simulink library "AFCToolbox2023a"  (R2023a)
settings: Solver=VariableStepAuto  StartTime=0.0  StopTime=10.0  RelTol=1e-3
undefined symbols (not defined in the file or in its folder): AFC5Toolbox_SimuMoudle, AFCToolbox, ax, ay, az, btnSample, C_d, C_dm, C_m, C_t, Control, d, declination_table, dp0, dp1, dp2, dp3, dt, euler_0, g0, I_xyz, inclination_table, J_m, lmd_high, lmd_low, lp_acc_knoise, lp_acc_max, lp_acc_min, lp_acc_seed, lp_GPS_BL_max, lp_GPS_BL_min, lp_GPS_H_max, lp_GPS_H_min, lp_GPS_knoise, lp_GPS_seed, lp_GPS_vel_max, lp_GPS_vel_min, lp_gyro_knoise, lp_gyro_max, lp_gyro_min, lp_gyro_seed, lp_hf_vwind, lp_hs_vwind_interp, lp_kaerorho, lp_kaeroT, lp_kIxyz, lp_kmass, lp_momentx_A0, lp_momentx_Af, lp_momentx_ts, lp_momenty_A0, lp_momenty_Af, lp_momenty_ts, lp_momentz_A0, lp_momentz_Af, lp_momentz_ts, lp_vf_vwind, lp_vs_vwind_interp, lp_vwind_thetax, lp_vwind_thetaz ... (+54)
libraries: $bdroot x104, simulink x75, etargetslib x32, sharedtransform x13, simulink_extras x12, dspstat3 x11, aerolibconvert2 x9, aerolibtransform2 x3, aerolibutil x2, matrix_library x1
(part 8 of 10)

== matlab function AFCToolbox2023a/ServoCardModule/XSrvoSamp/MATLAB Function ==
  data: ID1 input; out1 output; angleACK1 input; ID2 input; angleACK2 input; ID3 input; angleACK3 input; ID4 input; angleACK4 input; out2 output; out3 output; out4 output
function [out1, out2, out3, out4] = routeByID(ID1, angleACK1, ID2, angleACK2, ID3, angleACK3, ID4, angleACK4)
    % 1. 初始化输出数组（4个元素，对应Mux1-4号端口，默认0）
    out_array = zeros(1, 4);  % [out1, out2, out3, out4]
    
    % 2. 打包所有ID和angleACK为数组（批量处理，避免重复代码）
    IDs = [ID1, ID2, ID3, ID4];          % 所有ID的数组
    angles = [angleACK1, angleACK2, angleACK3, angleACK4];  % 所有角度的数组
    
    % 3. 循环遍历：ID在1-4范围内才赋值（索引直接对应端口）
    for i = 1:4
        id = IDs(i);
        if id >= 1 && id <= 4  % 仅处理合法ID（1-4）
            out_array(id) = angles(i);  % 关键：ID=1→out_array(1)=out1，直接索引赋值！
        end
    end
    
    % 4. 拆分输出数组为4个端口（对应Mux1-4号）
    [out1, out2, out3, out4] = deal(out_array(1), out_array(2), out_array(3), out_array(4));
end

== matlab function AFCToolbox2023a/SimuMoudle/Position-Control/Consistent formation control /一致性控制——F2/MATLAB Function1 ==
  data: r input; result output
function result = Faixy(r)
%UNTITLED 此处显示有关此函数的摘要


result=-1.8*(1-exp(-0.5*r))/(1+exp(-0.5*r));



end

== matlab function AFCToolbox2023a/SimuMoudle/Position-Control/Consistent formation control /一致性控制——F3/MATLAB Function2 ==
  data: r input; result output
function result = Faixy(r)
%UNTITLED 此处显示有关此函数的摘要


result=-1.8*(1-exp(-0.5*r))/(1+exp(-0.5*r));



end

== matlab function AFCToolbox2023a/SimuMoudle/Position-Control/Consistent formation control /一致性控制——F1/Subsystem1/MATLAB Function ==
  data: i input; wx output; dt input; wy output
function [wx,wy] = w_error(i,dt)
%W_ERROR 此处显示有关此函数的摘要
%   此处显示详细说明
wx = 0.1*(cos(i*dt+pi/6)+cos(i*dt/3+pi/6)+cos(i*dt/5+pi/6)+cos(i*dt/7+pi/6));
wy = 0.1*(sin(i*dt+pi/6)+sin(i*dt/3+pi/6)+sin(i*dt/5+pi/6)+sin(i*dt/7+pi/6));

end

== matlab function AFCToolbox2023a/SimuMoudle/Position-Control/Consistent formation control /一致性控制——F2/Subsystem2/MATLAB Function ==
  data: i input; wx output; dt input; wy output
function [wx,wy] = w_error(i,dt)
%W_ERROR 此处显示有关此函数的摘要
%   此处显示详细说明
wx = 0.1*(cos(i*dt+pi/6)+cos(i*dt/3+pi/6)+cos(i*dt/5+pi/6)+cos(i*dt/7+pi/6));
wy = 0.1*(sin(i*dt+pi/6)+sin(i*dt/3+pi/6)+sin(i*dt/5+pi/6)+sin(i*dt/7+pi/6));

end

== matlab function AFCToolbox2023a/SimuMoudle/Position-Control/Consistent formation control /一致性控制——F3/Subsystem1/MATLAB Function ==
  data: i input; wx output; dt input; wy output
function [wx,wy] = w_error(i,dt)
%W_ERROR 此处显示有关此函数的摘要
%   此处显示详细说明
wx = 0.1*(cos(i*dt+pi/6)+cos(i*dt/3+pi/6)+cos(i*dt/5+pi/6)+cos(i*dt/7+pi/6));
wy = 0.1*(sin(i*dt+pi/6)+sin(i*dt/3+pi/6)+sin(i*dt/5+pi/6)+sin(i*dt/7+pi/6));

end

== matlab function AFCToolbox2023a/SimuMoudle/Position-Control/Consistent formation control /一致性控制——F2/MATLAB Function2 ==
  data: r input; result output
function result = Faixy(r)
%UNTITLED 此处显示有关此函数的摘要


result=-1.8*(1-exp(-0.5*r))/(1+exp(-0.5*r));



end

== matlab function AFCToolbox2023a/SimuMoudle/Position-Control/Consistent formation control /一致性控制——F1/MATLAB Function1 ==
  data: r input; result output
function result = Faixy(r)
%UNTITLED 此处显示有关此函数的摘要


result=-1.8*(1-exp(-0.5*r))/(1+exp(-0.5*r));



end

== matlab function AFCToolbox2023a/SimuMoudle/Position-Control/Consistent formation control /一致性控制——F1/MATLAB Function2 ==
  data: r input; result output
function result = Faixy(r)
%UNTITLED 此处显示有关此函数的摘要


result=-1.8*(1-exp(-0.5*r))/(1+exp(-0.5*r));



end

== matlab function AFCToolbox2023a/SimuMoudle/Position-Control/Consistent formation control /一致性控制——F1/MATLAB Function4 ==
  data: r input; result output
function result = Faixy(r)
%UNTITLED 此处显示有关此函数的摘要


result=-1.8*(1-exp(-0.5*r))/(1+exp(-0.5*r));



end

== matlab function AFCToolbox2023a/SimuMoudle/Position-Control/Consistent formation control /一致性控制——F3/MATLAB Function3 ==
  data: r input; result output
function result = Faixy(r)
%UNTITLED 此处显示有关此函数的摘要


result=-1.8*(1-exp(-0.5*r))/(1+exp(-0.5*r));



end

== matlab function AFCToolbox2023a/SimuMoudle/Position-Control/Leader/Subsystem/Follower1/MATLAB Function ==
  data: theta input; J output; phi input; v input
function J = TA_xyz(theta,phi,v)
a=cos(theta)*cos(phi);
b=-v*sin(theta)*cos(phi);
c=-v*cos(theta)*sin(phi);

d=sin(theta)*cos(phi);
e=v*cos(theta)*cos(phi);
f=-v*sin(theta)*sin(phi);

g=sin(phi);
h=0;
i=v*cos(phi);

J=[a,b,c;
    d,e,f;
    g,h,i];
end

== matlab function AFCToolbox2023a/SimuMoudle/Position-Control/Leader/Subsystem/Follower1/MATLAB Function1 ==
  data: W input; result output
function result = Faiv(W)
%UNTITLED 此处显示有关此函数的摘要


result=-0.5*(1-exp(-0.5*W))/(1+exp(-0.5*W));



end

== matlab function AFCToolbox2023a/SimuMoudle/Position-Control/Leader/Subsystem/Follower1/MATLAB Function2 ==
  data: w input; result output
function result = Faiv(w)
%UNTITLED 此处显示有关此函数的摘要


result=-0.5*(1-exp(-0.5*w))/(1+exp(-0.5*w));



end

== matlab function AFCToolbox2023a/SimuMoudle/Position-Control/Leader/Subsystem/Follower1/MATLAB Function3 ==
  data: r input; result output
function result = Faiv(r)
%UNTITLED 此处显示有关此函数的摘要


result=-0.5*(1-exp(-0.5*r))/(1+exp(-0.5*r));



end

== matlab function AFCToolbox2023a/SimuMoudle/Position-Control/Leader/Subsystem/Follower2/MATLAB Function ==
  data: theta input; J output; phi input; v input
function J = TA_xyz(theta,phi,v)
a=cos(theta)*cos(phi);
b=-v*sin(theta)*cos(phi);
c=-v*cos(theta)*sin(phi);

d=sin(theta)*cos(phi);
e=v*cos(theta)*cos(phi);
f=-v*sin(theta)*sin(phi);

g=sin(phi);
h=0;
i=v*cos(phi);

J=[a,b,c;
    d,e,f;
    g,h,i];
end

== matlab function AFCToolbox2023a/SimuMoudle/Position-Control/Leader/Subsystem/Follower2/MATLAB Function1 ==
  data: W input; result output
function result = Faiv(W)
%UNTITLED 此处显示有关此函数的摘要


result=-0.5*(1-exp(-0.5*W))/(1+exp(-0.5*W));



end

== matlab function AFCToolbox2023a/SimuMoudle/Position-Control/Leader/Subsystem/Follower2/MATLAB Function2 ==
  data: w input; result output
function result = Faiv(w)
%UNTITLED 此处显示有关此函数的摘要


result=-0.5*(1-exp(-0.5*w))/(1+exp(-0.5*w));



end

== matlab function AFCToolbox2023a/SimuMoudle/Position-Control/Leader/Subsystem/Follower2/MATLAB Function3 ==
  data: r input; result output
function result = Faiv(r)
%UNTITLED 此处显示有关此函数的摘要


result=-0.5*(1-exp(-0.5*r))/(1+exp(-0.5*r));



end

== matlab function AFCToolbox2023a/SimuMoudle/Position-Control/Leader/Subsystem/Follower3/MATLAB Function ==
  data: theta input; J output; phi input; v input
function J = TA_xyz(theta,phi,v)
a=cos(theta)*cos(phi);
b=-v*sin(theta)*cos(phi);
c=-v*cos(theta)*sin(phi);

d=sin(theta)*cos(phi);
e=v*cos(theta)*cos(phi);
f=-v*sin(theta)*sin(phi);

g=sin(phi);
h=0;
i=v*cos(phi);

J=[a,b,c;
    d,e,f;
    g,h,i];
end

== matlab function AFCToolbox2023a/SimuMoudle/Position-Control/Leader/Subsystem/Follower3/MATLAB Function1 ==
  data: W input; result output
function result = Faiv(W)
%UNTITLED 此处显示有关此函数的摘要


result=-0.5*(1-exp(-0.5*W))/(1+exp(-0.5*W));



end

== stateflow chart AFCToolbox2023a/SimuMoudle/UAV/Equations of Motion/Chart ==
  state Land
    en, du: ground_contact = 1;
  state Flight
    en, du: ground_contact = 0;
  (default) -> Land
  Flight -> Land : [h<=0 && vel(3) >0]
  Land -> Flight : [acc(3)<0]
  data: h input; vel input; acc input; ground_contact output

== matlab function AFCToolbox2023a/SimuMoudle/Position-Control/Leader/Subsystem/Follower3/MATLAB Function2 ==
  data: w input; result output
function result = Faiv(w)
%UNTITLED 此处显示有关此函数的摘要


result=-0.5*(1-exp(-0.5*w))/(1+exp(-0.5*w));



end

== matlab function AFCToolbox2023a/SimuMoudle/Position-Control/Leader/Subsystem/Follower3/MATLAB Function3 ==
  data: r input; result output
function result = Faiv(r)
%UNTITLED 此处显示有关此函数的摘要


result=-0.5*(1-exp(-0.5*r))/(1+exp(-0.5*r));



end

== matlab function AFCToolbox2023a/SimuMoudle/SimuGps/LLA model/Subsystem1/ECEF地心坐标系-经纬高 ==
  data: x input; l output; y input; z input; b output; h output
function [l,b,h] = fcn(x,y,z)
[l,b,h] = xyz2lbh(x,y,z);

== matlab function AFCToolbox2023a/SimuMoudle/Position-Control/Consistent formation control /一致性控制——F3/MATLAB Function1 ==
  data: r input; result output
function result = Faixy(r)
%UNTITLED 此处显示有关此函数的摘要


result=-1.8*(1-exp(-0.5*r))/(1+exp(-0.5*r));



end

== matlab function AFCToolbox2023a/SimuMoudle/SimuGps/LLA model/Subsystem1/北天东-ECEF地心坐标系 ==
  data: pn input; DX output; ph input; pe input; Lon0 input; Lat0 input; Alt0 input; DY output; DZ output
function [ DX,DY,DZ ] = TransformBTD_T_DX( pn,ph,pe,Lon0,Lat0,Alt0 )
%TransformBTDTDX 此处显示有关此函数的摘要
%将北天东系转换到地心坐标系
m_dN_LE = zeros(3,3);

[ DX0,DY0,DZ0 ] = TransformLLA_T_DX(Lon0,Lat0,Alt0);%经纬高转为地面坐标系G

Fai = Lat0;
Lamda = Lon0;

x_bt = pn;
y_bt = ph;
z_bt = pe;

m_dN_LE(1,1) = -sin(Fai)*cos(Lamda);
m_dN_LE(1,2) = cos(Fai)*cos(Lamda);
m_dN_LE(1,3) = -sin(Lamda);
m_dN_LE(2,1) = -sin(Fai)*sin(Lamda);
m_dN_LE(2,2) = cos(Fai)*sin(Lamda);
m_dN_LE(2,3) = cos(Lamda);
m_dN_LE(3,1) = cos(Fai);
m_dN_LE(3,2) = sin(Fai);
m_dN_LE(3,3) = 0.0;

A = m_dN_LE*[x_bt;y_bt;z_bt];
x_dx = A(1);
y_dx = A(2);
z_dx = A(3);

DX = DX0 + x_dx;
DY = DY0 + y_dx;
DZ = DZ0 + z_dx;

end

== matlab function AFCToolbox2023a/SimuMoudle/SimuICM/acclerate  model2/Subsystem/MATLAB Function ==
  data: accBias input; accData output; correlationTimeConstant input; accNoiseStdDev input; dt input
function accData= fcn(accBias,correlationTimeConstant,accNoiseStdDev,dt)
persistent initaccBias;

%单位换算
arcdeg = pi/180;hur = 3600;dph = arcdeg / hur;Hz = 1;g=9.7803267714;
% accNoiseStdDev = 100;           % 加速度一阶马尔可夫噪声均方根ug
% accBiasOffsetStdDev =100;      % 陀螺仪零偏漂移标准差ug
% 
% %常值漂移
% eb = accBiasOffsetStdDev * g * randn(1,1);

%一阶马尔可夫相关时间T;反相关时间beta = 1/T;
% TauG = 3600;
beta = 1/correlationTimeConstant; 
% 方差R0（m/s^2）
R0 = (accNoiseStdDev*g)^2;

%角速率随机游走系数
q = 2*beta*R0;


if isempty(initaccBias)
    initaccBias = sqrt(R0)*randn(1,1);
    accBias= initaccBias;
end

 
Phi = 1 -beta*dt;
sQkr =sqrt(q*dt);
accBias=Phi*accBias+sQkr*randn(1,1);
% 生成加速度数据
accData =  accBias;
end

== matlab function AFCToolbox2023a/SimuMoudle/SimuICM/acclerate  model2/Subsystem1/MATLAB Function ==
  data: accBias input; accData output; correlationTimeConstant input; accNoiseStdDev input; dt input
function accData= fcn(accBias,correlationTimeConstant,accNoiseStdDev,dt)
persistent initaccBias;

%单位换算
arcdeg = pi/180;hur = 3600;dph = arcdeg / hur;Hz = 1;g=9.7803267714;
% accNoiseStdDev = 100;           % 加速度一阶马尔可夫噪声均方根ug
% accBiasOffsetStdDev =100;      % 陀螺仪零偏漂移标准差ug
% 
% %常值漂移
% eb = accBiasOffsetStdDev * g * randn(1,1);

%一阶马尔可夫相关时间T;反相关时间beta = 1/T;
% TauG = 3600;
beta = 1/correlationTimeConstant; 
% 方差R0（m/s^2）
R0 = (accNoiseStdDev*g)^2;

%角速率随机游走系数
q = 2*beta*R0;


if isempty(initaccBias)
    initaccBias = sqrt(R0)*randn(1,1);
    accBias= initaccBias;
end

 
Phi = 1 -beta*dt;
sQkr =sqrt(q*dt);
accBias=Phi*accBias+sQkr*randn(1,1);
% 生成加速度数据
accData =  accBias;
end

== matlab function AFCToolbox2023a/SimuMoudle/SimuICM/acclerate  model2/Subsystem2/MATLAB Function ==
  data: accBias input; accData output; correlationTimeConstant input; accNoiseStdDev input; dt input
function accData= fcn(accBias,correlationTimeConstant,accNoiseStdDev,dt)
persistent initaccBias;

%单位换算
arcdeg = pi/180;hur = 3600;dph = arcdeg / hur;Hz = 1;g=9.7803267714;
% accNoiseStdDev = 100;           % 加速度一阶马尔可夫噪声均方根ug
% accBiasOffsetStdDev =100;      % 陀螺仪零偏漂移标准差ug
% 
% %常值漂移
% eb = accBiasOffsetStdDev * g * randn(1,1);

%一阶马尔可夫相关时间T;反相关时间beta = 1/T;
% TauG = 3600;
beta = 1/correlationTimeConstant; 
% 方差R0（m/s^2）
R0 = (accNoiseStdDev*g)^2;

%角速率随机游走系数
q = 2*beta*R0;


if isempty(initaccBias)
    initaccBias = sqrt(R0)*randn(1,1);
    accBias= initaccBias;
end

 
Phi = 1 -beta*dt;
sQkr =sqrt(q*dt);
accBias=Phi*accBias+sQkr*randn(1,1);
% 生成加速度数据
accData =  accBias;
end

== matlab function AFCToolbox2023a/SimuMoudle/SimuICM/gyro model1/Subsystem/MATLAB Function ==
  data: gyroBias input; gyroData output; correlationTimeConstant input; gyroNoiseStdDev input; dt input
function gyroData= fcn(gyroBias,correlationTimeConstant,gyroNoiseStdDev,dt)
persistent initgyroBias;

%单位换算
arcdeg = pi/180;hur = 3600;dph = arcdeg / hur;Hz = 1;
% gyroNoiseStdDev = 0.1;           % 陀螺仪一阶马尔可夫噪声均方根°/h
% gyroBiasOffsetStdDev = 0.1;      % 陀螺仪零偏漂移标准差rad/s
% 
% %常值漂移
% eb = gyroBiasOffsetStdDev * dph * randn(1,1);

%一阶马尔可夫相关时间T;反相关时间beta = 1/T;
% TauG = 3600;
beta = 1/correlationTimeConstant; 
% 方差R0（rad/s）
R0 = (gyroNoiseStdDev*dph)^2;

%角速率随机游走系数
q = 2*beta*R0;


if isempty(initgyroBias)
    initgyroBias = sqrt(R0)*randn(1,1);
    gyroBias= initgyroBias;
end

 
Phi = 1 -beta*dt;
sQkr =sqrt(q*dt);
gyroBias=Phi*gyroBias+sQkr*randn(1,1);
% 生成陀螺仪数据
gyroData =  gyroBias;
end

== matlab function AFCToolbox2023a/SimuMoudle/SimuICM/gyro model1/Subsystem1/MATLAB Function ==
  data: gyroBias input; gyroData output; correlationTimeConstant input; gyroNoiseStdDev input; dt input
function gyroData= fcn(gyroBias,correlationTimeConstant,gyroNoiseStdDev,dt)
persistent initgyroBias;

%单位换算
arcdeg = pi/180;hur = 3600;dph = arcdeg / hur;Hz = 1;
% gyroNoiseStdDev = 0.1;           % 陀螺仪一阶马尔可夫噪声均方根°/h
% gyroBiasOffsetStdDev = 0.1;      % 陀螺仪零偏漂移标准差rad/s
% 
% %常值漂移
% eb = gyroBiasOffsetStdDev * dph * randn(1,1);

%一阶马尔可夫相关时间T;反相关时间beta = 1/T;
% TauG = 3600;
beta = 1/correlationTimeConstant; 
% 方差R0（rad/s）
R0 = (gyroNoiseStdDev*dph)^2;

%角速率随机游走系数
q = 2*beta*R0;


if isempty(initgyroBias)
    initgyroBias = sqrt(R0)*randn(1,1);
    gyroBias= initgyroBias;
end

 
Phi = 1 -beta*dt;
sQkr =sqrt(q*dt);
gyroBias=Phi*gyroBias+sQkr*randn(1,1);
% 生成陀螺仪数据
gyroData =  gyroBias;
end

== matlab function AFCToolbox2023a/SimuMoudle/Position-Control/Leader/MATLAB Function ==
  data: theta input; J output; phi input; v input
function J = TA_xyz(theta,phi,v)
a=cos(theta)*cos(phi);
b=-v*sin(theta)*cos(phi);
c=-v*cos(theta)*sin(phi);

d=sin(theta)*cos(phi);
e=v*cos(theta)*cos(phi);
f=-v*sin(theta)*sin(phi);

g=sin(phi);
h=0;
i=v*cos(phi);

J=[a,b,c;
    d,e,f;
    g,h,i];
end

== matlab function AFCToolbox2023a/SimuMoudle/SimuICM/gyro model1/Subsystem2/MATLAB Function ==
  data: gyroBias input; gyroData output; correlationTimeConstant input; gyroNoiseStdDev input; dt input
function gyroData= fcn(gyroBias,correlationTimeConstant,gyroNoiseStdDev,dt)
persistent initgyroBias;

%单位换算
arcdeg = pi/180;hur = 3600;dph = arcdeg / hur;Hz = 1;
% gyroNoiseStdDev = 0.1;           % 陀螺仪一阶马尔可夫噪声均方根°/h
% gyroBiasOffsetStdDev = 0.1;      % 陀螺仪零偏漂移标准差rad/s
% 
% %常值漂移
% eb = gyroBiasOffsetStdDev * dph * randn(1,1);

%一阶马尔可夫相关时间T;反相关时间beta = 1/T;
% TauG = 3600;
beta = 1/correlationTimeConstant; 
% 方差R0（rad/s）
R0 = (gyroNoiseStdDev*dph)^2;

%角速率随机游走系数
q = 2*beta*R0;


if isempty(initgyroBias)
    initgyroBias = sqrt(R0)*randn(1,1);
    gyroBias= initgyroBias;
end

 
Phi = 1 -beta*dt;
sQkr =sqrt(q*dt);
gyroBias=Phi*gyroBias+sQkr*randn(1,1);
% 生成陀螺仪数据
gyroData =  gyroBias;
end

== matlab function AFCToolbox2023a/SimuMoudle/SimuBaro/Baro model/MATLAB Function ==
  data: h input; P output
function P = altitude_to_pressure(h)
    % 输入：高度 h（单位：米）
    % 输出：压强 P（单位：Pa）

    % 常量定义
    P0 = 101325;  % 海平面上的大气压强，单位Pa
    L = 0.0065;   % 温度递减率，单位K/m
    T0 = 288.15;  % 海平面上的温度，单位K
    g0 = 9.80665; % 重力加速度，单位m/s²
    M = 0.0289644; % 空气摩尔质量，单位kg/mol
    R = 8.314462618; % 气体常数，单位J/(mol·K)

    % 计算压强
    P = P0 * (1 - (L * h) / T0)^(g0 * M / (R * L));
end

== matlab function AFCToolbox2023a/SimuMoudle/SimuBaro/Baro model/MATLAB Function1 ==
  data: altitude input; pressure output; temperature output
function [pressure, temperature] = calculateAtmosphereProperties(altitude)
    % 标准大气参数
    R = 287; % 干空气的特定气体常数，单位 J/(kg*K)
    g = 9.81; % 重力加速度，单位 m/s^2
    T0 = 293.15; % 海平面标准温度，单位 K
    p0 = 101325; % 海平面标准压强，单位 Pa
    lapserate = -0.0065; % 环境递减率，单位 K/m

    % 计算给定高度的压强和温度
    if altitude <= 11000
        temperature = T0 + lapserate * altitude; % 温度随高度线性递减
    else
        temperature = T0 + lapserate * 11000; % 高于11公里后温度保持不变
    end
    pressure = p0 * (T0/temperature)^(-g/R/lapserate); % 压强随高度和温度变化

    % 输出结果
    pressure = pressure; % 返回压强
    
    % 将温度从开尔文转换为摄氏度
    temperature = temperature - 273.15;% 返回温度
end

== matlab function AFCToolbox2023a/基础导航算法模型库/ECL EKF/Subsystem/InitCovariance1 ==
  data: covariance output; dt input
function covariance = InitCovariance(dt)
%% Initial Uncertainty
param.alignment.posErrNE = 10.0; % Initial 1SD position error when aligning without GPS. (m/sec)
param.alignment.velErrNE = 5.0; % Initial 1SD velocity error when aligning without GPS. (m/sec)
param.alignment.velErrD = 1.0; % Initial 1SD vertical velocity error when aligning without GPS. (m/sec)
param.alignment.delAngBiasErr = 0.05*pi/180; % Initial 1SD rate gyro bias uncertainty. (rad/sec)
param.alignment.delVelBiasErr = 0.07; % Initial 1SD accelerometer bias uncertainty. (m/sec^2)
param.alignment.quatErr = 0.01; % Initial 1SD uncertainty in quaternion.
param.alignment.magErrXYZ = 0.01; % Initial 1SD uncertainty in body frame XYZ magnetic field states. (gauss)
param.alignment.magErrNED = 0.5; % Initial 1SD uncertainty in earth frame NED magnetic field states. (gauss)
param.alignment.hgtErr = 0.5; % Initial 1SD uncertainty in height. (m)
param.alignment.windErrNE = 5.0; % Initial 1SD error in wind states. (m/sec)


% Define quaternion state errors
Sigma_quat = param.alignment.quatErr * [1;1;1;1];
% Define velocity state errors
Sigma_velocity = param.alignment.velErrNE * [1;1;1];

% Define position state errors
Sigma_position = param.alignment.posErrNE * [1;1;1];


% Define delta angle bias state errors
Sigma_dAngBias = param.alignment.delAngBiasErr*dt*[1;1;1];

% Define delta velocity bias state errors
Sigma_dVelBias = param.alignment.delVelBiasErr*dt*[1;1;1];

% Define magnetic field state errors
Sigma_magNED = [param.alignment.magErrNED;param.alignment.magErrNED;param.alignment.magErrNED]; % 1 Sigma uncertainty in initial NED mag field
Sigma_magXYZ = [param.alignment.magErrXYZ;param.alignment.magErrXYZ;param.alignment.magErrXYZ]; % 1 Sigma uncertainty in initial XYZ mag sensor offset

% Define wind velocity state errors
Sigma_wind = param.alignment.windErrNE * [1;1];

% Convert to variances and write to covariance matrix diagonals
covariance = diag([Sigma_quat;Sigma_velocity;Sigma_position;Sigma_dAngBias;Sigma_dVelBias;Sigma_magNED;Sigma_magXYZ;Sigma_wind].^2);
end

== matlab function AFCToolbox2023a/基础导航算法模型库/ECL EKF/Subsystem/Mag Fusion/Control MagDeclination Fusion1 ==
  data: states input; states output; P input; R_decl input; measDec input; P output
function [...
    states, ... % state vector after fusion of measurements
    P] ... %
    = FuseMagDeclination( ...
    states, ... % state vector after fusion of measurements
    P, ... %
    R_decl,...
    measDec) % magnetic field declination - azimuth angle measured from true north (rad)

% magNE
magN = states(17);
magE = states(18);

H = zeros(1,24);
Kfusion = zeros(24,1);

R_DECL = R_decl^2;
	HK0 = power(magN, -2);
	HK1 = HK0*power(magE, 2) + 1.0;
	HK2 = 1.0/HK1;
	HK3 = 1.0/magN;
	HK4 = HK2*HK3;
    HK5 = HK3*magE;
	HK6 = HK5*P(17,18) - P(18,18);
	HK7 = power(HK1, -2);
	HK8 = HK5*P(17,17) - P(17,18);
    innovation_variance = -HK0*HK6*HK7 + HK7*HK8*magE/power(magN, 3) + R_DECL;
    HK9 = HK4/innovation_variance;

H(17) = -HK0*HK2*magE;
H(18) = HK4;

	for row = 1:16
		Kfusion(row) = -HK9*(HK5*P(row,17) - P(row,18));
    end

	Kfusion(17) = -HK8*HK9;
	Kfusion(18) = -HK6*HK9;

	for  row = 19:24
		Kfusion(row) = -HK9*(HK5*P(17,row) - P(18,row));
    end


% Magnetic declination noise R = σdelc^2
%R_MAG = 0.5^2;

%% Hψ_dec = ∂ψ_dec / ∂x
%H = calcH_MAGD(magE,magN);
% S = Hψ_dec * P * PT + R_MAG
%varInnov = (H*P*transpose(H) + R_MAG);
% Optimal Kalman gain, K = Pk+1|k * Hψ_dec / S
%Kfusion = (P*transpose(H))/varInnov;

% Calculate the predicted magnetic declination, ψ_dec = arctan(mE/mN)
predDec = atan2(magE,magN);

% Calculate the measurement innovation, yk = zψ_dec - ψ_dec
innovation = measDec- predDec;

if (innovation > 0.5)
    innovation = single(0.5);
elseif (innovation < -0.5)
    innovation = single(-0.5);
end

% correct the state vector, xk+1|k+1 = xk+1|k + K*yk
states = states + Kfusion * innovation;

% correct the covariance Pk+1|k+1 = Pk+1|k - K * Hψ_dec * Pk+1|k
%P = P - Kfusion*H*P;
KHP = computeKHP(Kfusion, H, P);
P = P - KHP;
%% Force symmetry on the covariance matrix to prevent ill-conditioning
% of the matrix which would cause the filter to blow-up
P = 0.5*(P + transpose(P));

% ensure diagonals are positive
for i=1:24
    if P(i,i) < 0
        P(i,i) = single(0);
    end
end
% fixCovarianceErrors(true);
% limitDeclination();
end

== matlab function AFCToolbox2023a/基础导航算法模型库/ECL EKF/Subsystem/Mag Fusion/Control Magneto meter Fusion2 ==
  data: fault_status_flags_bad_mag output; states input; states output; P input; Measmag input; R_MAG input; P output
function [fault_status_flags_bad_mag,...
    states, ... % state vector after fusion of measurements
    P] ...% state covariance matrix after fusion of corrections
    = FuseMagnetometer( ...
    states, ... % predicted states
    P, ... % predicted covariance
    Measmag, ... % body frame magnetic flux measurements
    R_MAG) % magnetometer measurement variance - gauss^2
   
% control.cpp -> controlMagFusion()
% ~ mag_control.cpp -> controlMagFusion() -> runMagAndMagDeclFusions(...)-> 
% ~ mag_fusion.cpp -> fuseMag(...) -> fuseDeclination(...)
fault_status_flags_bad_mag = zeros(1,3);
% assign intermediate variables

% quaternion
q0 = states(1);
q1 = states(2);
q2 = states(3);
q3 = states(4);
% magnetometer bais
magXbias = states(20);
magYbias = states(21);
magZbias = states(22);
mag_B = [magXbias;magYbias;magZbias];
% magNED
magN = states(17);
magE = states(18);
magD = states(19);


% XYZ Measurement uncertainty. Need to consider timing errors for fast rotations
% R_MAG = power(max(params_mag_noise, 0.0),2);
mag_innov_var = zeros(1,3);

% calculate intermediate variables used for X axis innovation variance, observation Jacobians and Kalman gains
% const char* numerical_error_covariance_reset_string = "numerical error - covariance reset";
HKX0 = -magD*q2 + magE*q3 + magN*q0;
HKX1 = magD*q3 + magE*q2 + magN*q1;
HKX2 = magE*q1;
HKX3 = magD*q0;
HKX4 = magN*q2;
HKX5 = magD*q1 + magE*q0 - magN*q3;
HKX6 = power(q0, 2) + power(q1, 2) - power(q2, 2) - power(q3, 2);
HKX7 = q0*q3 + q1*q2;
HKX8 = q1*q3;
HKX9 = q0*q2;
HKX10 = 2*HKX7;
HKX11 = -2*HKX8 + 2*HKX9;
HKX12 = 2*HKX1;
HKX13 = 2*HKX0;
HKX14 = -2*HKX2 + 2*HKX3 + 2*HKX4;
HKX15 = 2*HKX5;
HKX16 = HKX10*P(1,18) - HKX11*P(1,19) + HKX12*P(1,2) + HKX13*P(1,1) - HKX14*P(1,3) + HKX15*P(1,4) + HKX6*P(1,17) + P(1,20);
HKX17 = HKX10*P(17,18) - HKX11*P(17,19) + HKX12*P(2,17) + HKX13*P(1,17) - HKX14*P(3,17) + HKX15*P(4,17) + HKX6*P(17,17) + P(17,18);
HKX18 = HKX10*P(18,19) - HKX11*P(19,19) + HKX12*P(2,19) + HKX13*P(1,19) - HKX14*P(3,19) + HKX15*P(4,19) + HKX6*P(17,19) + P(19,20);
HKX19 = HKX10*P(3,18) - HKX11*P(3,19) + HKX12*P(2,3) + HKX13*P(1,3) - HKX14*P(3,3) + HKX15*P(3,4) + HKX6*P(3,17) + P(3,20);
HKX20 = HKX10*P(18,18) - HKX11*P(18,19) + HKX12*P(2,18) + HKX13*P(1,18) - HKX14*P(3,18) + HKX15*P(4,18) + HKX6*P(17,18) + P(18,20);
HKX21 = HKX10*P(4,18) - HKX11*P(4,19) + HKX12*P(2,4) + HKX13*P(1,4) - HKX14*P(3,4) + HKX15*P(4,4) + HKX6*P(4,17) + P(4,20);
HKX22 = HKX10*P(2,18) - HKX11*P(2,19) + HKX12*P(2,2) + HKX13*P(1,2) - HKX14*P(2,3) + HKX15*P(2,4) + HKX6*P(2,17) + P(2,20);
HKX23 = HKX10*P(18,20) - HKX11*P(19,20) + HKX12*P(2,20) + HKX13*P(1,20) - HKX14*P(3,20) + HKX15*P(4,20) + HKX6*P(17,20) + P(20,20);

mag_innov_var(1) = HKX10*HKX20 - HKX11*HKX18 + HKX12*HKX22 + HKX13*HKX16 - HKX14*HKX19 + HKX15*HKX21 + HKX17*HKX6 + HKX23 + R_MAG;

if (mag_innov_var(1) < R_MAG) 
	% the innovation variance contribution from the state covariances is negative which means the covariance matrix is badly conditioned
	fault_status_flags_bad_mag_x = 1;

	% we need to re-initialise covariances and abort this fusion step
	% resetMagRelatedCovariances();
    P = resetMagRelatedCovariances(P,states);
    return;
end
fault_status_flags_bad_mag_x = 0;
% fault_status_flags_bad_mag_x = false;

HKX24 = 1.0/mag_innov_var(1);

% intermediate variables for calculation of innovations variances for Y and Z axes
% don't calculate all terms needed for observation jacobians and Kalman gains because
% these will have to be recalculated when the X and Y axes are fused
IV0 = q0*q1;
IV1 = q2*q3;
IV2 = 2*IV0 + 2*IV1;
IV3 = 2*q0*q3 - 2*q1*q2;
IV4 = 2*magD*q3 + 2*magE*q2 + 2*magN*q1;
IV5 = 2*magD*q1 + 2*magE*q0 - 2*magN*q3;
IV6 = 2*magD*q0 - 2*magE*q1 + 2*magN*q2;
IV7 = -2*magD*q2 + 2*magE*q3 + 2*magN*q0;
IV8 = power(q2, 2);
IV9 = power(q3, 2);
IV10 = power(q0, 2) - power(q1, 2);
IV11 = IV10 + IV8 - IV9;
% const float IV12 = IV7*P(2,3);
% const float IV13 = IV5*P(0,1);
% const float IV14 = IV6*P(0,1);
% const float IV15 = IV4*P(2,3);
IV12 = IV7*P(3,4);
IV13 = IV5*P(1,2);
IV14 = IV6*P(1,2);
IV15 = IV4*P(3,4);
IV16 = 2*q0*q2 + 2*q1*q3;
IV17 = 2*IV0 - 2*IV1;
IV18 = IV10 - IV8 + IV9;
% _mag_innov_var(1) = IV11*P(17,20) + IV11*(IV11*P(17,17) + IV2*P(17,18) - IV3*P(16,17) + IV4*P(2,17) + IV5*P(0,17) + IV6*P(1,17) - IV7*P(3,17) + P(17,20)) + IV2*P(18,20) + IV2*(IV11*P(17,18) + IV2*P(18,18) - IV3*P(16,18) + IV4*P(2,18) + IV5*P(0,18) + IV6*P(1,18) - IV7*P(3,18) + P(18,20)) - IV3*P(16,20) - IV3*(IV11*P(16,17) + IV2*P(16,18) - IV3*P(16,16) + IV4*P(2,16) + IV5*P(0,16) + IV6*P(1,16) - IV7*P(3,16) + P(16,20)) + IV4*P(2,20) + IV4*(IV11*P(2,17) - IV12 + IV2*P(2,18) - IV3*P(2,16) + IV4*P(2,2) + IV5*P(0,2) + IV6*P(1,2) + P(2,20)) + IV5*P(0,20) + IV5*(IV11*P(0,17) + IV14 + IV2*P(0,18) - IV3*P(0,16) + IV4*P(0,2) + IV5*P(0,0) - IV7*P(0,3) + P(0,20)) + IV6*P(1,20) + IV6*(IV11*P(1,17) + IV13 + IV2*P(1,18) - IV3*P(1,16) + IV4*P(1,2) + IV6*P(1,1) - IV7*P(1,3) + P(1,20)) - IV7*P(3,20) - IV7*(IV11*P(3,17) + IV15 + IV2*P(3,18) - IV3*P(3,16) + IV5*P(0,3) + IV6*P(1,3) - IV7*P(3,3) + P(3,20)) + P(20,20) + R_MAG;
mag_innov_var(2) = IV11*P(18,21) + IV11*(IV11*P(18,18) + IV2*P(18,19) - IV3*P(17,18) + IV4*P(3,18) + IV5*P(1,18) + IV6*P(2,18) - IV7*P(4,18) + P(18,21)) + IV2*P(19,21) + IV2*(IV11*P(18,19) + IV2*P(19,19) - IV3*P(17,19) + IV4*P(3,19) + IV5*P(1,19) + IV6*P(2,19) - IV7*P(4,19) + P(19,21)) - IV3*P(17,21) - IV3*(IV11*P(17,18) + IV2*P(17,19) - IV3*P(17,17) + IV4*P(3,17) + IV5*P(1,17) + IV6*P(2,17) - IV7*P(4,17) + P(17,21)) + IV4*P(3,21) + IV4*(IV11*P(3,18) - IV12 + IV2*P(3,19) - IV3*P(3,17) + IV4*P(3,3) + IV5*P(1,3) + IV6*P(2,3) + P(3,21)) + IV5*P(1,21) + IV5*(IV11*P(1,18) + IV14 + IV2*P(1,19) - IV3*P(1,17) + IV4*P(1,3) + IV5*P(1,1) - IV7*P(1,4) + P(1,21)) + IV6*P(2,21) + IV6*(IV11*P(2,18) + IV13 + IV2*P(2,19) - IV3*P(2,17) + IV4*P(2,3) + IV6*P(2,2) - IV7*P(2,4) + P(2,21)) - IV7*P(4,21) - IV7*(IV11*P(4,18) + IV15 + IV2*P(4,19) - IV3*P(4,17) + IV5*P(1,4) + IV6*P(2,4) - IV7*P(4,4) + P(4,21)) + P(21,21) + R_MAG;
% _mag_innov_var(2) = IV16*P(16,21) + IV16*(IV16*P(16,16) - IV17*P(16,17) + IV18*P(16,18) + IV4*P(3,16) - IV5*P(1,16) + IV6*P(0,16) + IV7*P(2,16) + P(16,21)) - IV17*P(17,21) - IV17*(IV16*P(16,17) - IV17*P(17,17) + IV18*P(17,18) + IV4*P(3,17) - IV5*P(1,17) + IV6*P(0,17) + IV7*P(2,17) + P(17,21)) + IV18*P(18,21) + IV18*(IV16*P(16,18) - IV17*P(17,18) + IV18*P(18,18) + IV4*P(3,18) - IV5*P(1,18) + IV6*P(0,18) + IV7*P(2,18) + P(18,21)) + IV4*P(3,21) + IV4*(IV12 + IV16*P(3,16) - IV17*P(3,17) + IV18*P(3,18) + IV4*P(3,3) - IV5*P(1,3) + IV6*P(0,3) + P(3,21)) - IV5*P(1,21) - IV5*(IV14 + IV16*P(1,16) - IV17*P(1,17) + IV18*P(1,18) + IV4*P(1,3) - IV5*P(1,1) + IV7*P(1,2) + P(1,21)) + IV6*P(0,21) + IV6*(-IV13 + IV16*P(0,16) - IV17*P(0,17) + IV18*P(0,18) + IV4*P(0,3) + IV6*P(0,0) + IV7*P(0,2) + P(0,21)) + IV7*P(2,21) + IV7*(IV15 + IV16*P(2,16) - IV17*P(2,17) + IV18*P(2,18) - IV5*P(1,2) + IV6*P(0,2) + IV7*P(2,2) + P(2,21)) + P(21,21) + R_MAG;
mag_innov_var(3) = IV16*P(17,22) + IV16*(IV16*P(17,17) - IV17*P(17,18) + IV18*P(17,19) + IV4*P(4,17) - IV5*P(2,17) + IV6*P(1,17) + IV7*P(3,17) + P(17,22)) - IV17*P(18,22) - IV17*(IV16*P(17,18) - IV17*P(18,18) + IV18*P(18,19) + IV4*P(4,18) - IV5*P(2,18) + IV6*P(1,18) + IV7*P(3,18) + P(18,22)) + IV18*P(19,22) + IV18*(IV16*P(17,19) - IV17*P(18,19) + IV18*P(19,19) + IV4*P(4,19) - IV5*P(2,19) + IV6*P(1,19) + IV7*P(3,19) + P(19,22)) + IV4*P(4,22) + IV4*(IV12 + IV16*P(4,17) - IV17*P(4,18) + IV18*P(4,19) + IV4*P(4,4) - IV5*P(2,4) + IV6*P(1,4) + P(4,22)) - IV5*P(2,22) - IV5*(IV14 + IV16*P(2,17) - IV17*P(2,18) + IV18*P(2,19) + IV4*P(2,4) - IV5*P(2,2) + IV7*P(2,3) + P(2,22)) + IV6*P(1,22) + IV6*(-IV13 + IV16*P(1,17) - IV17*P(1,18) + IV18*P(1,19) + IV4*P(1,4) + IV6*P(1,1) + IV7*P(1,3) + P(1,22)) + IV7*P(3,22) + IV7*(IV15 + IV16*P(3,17) - IV17*P(3,18) + IV18*P(3,19) - IV5*P(2,3) + IV6*P(1,3) + IV7*P(3,3) + P(3,22)) + P(22,22) + R_MAG;

% chedk innovation variances for being badly conditioned
if (mag_innov_var(2) < R_MAG) 
	% the innovation variance contribution from the state covariances is negtive which means the covariance matrix is badly conditioned
	fault_status_flags_bad_mag_y = 1;

	% we need to re-initialise covariances and abort this fusion step
	% resetMagRelatedCovariances();
    P = resetMagRelatedCovariances(P,states);
    return;
end
fault_status_flags_bad_mag_y = 0;
% fault_status_flags_bad_mag_y = false;

if (mag_innov_var(3) < R_MAG) 
	% the innovation variance contribution from the state covariances is negative which means the covariance matrix is badly conditioned
	fault_status_flags_bad_mag_z = 1;

	% we need to re-initialise covariances and abort this fusion step
	% resetMagRelatedCovariances();
    P = resetMagRelatedCovariances(P,states);
    return;
end
fault_status_flags_bad_mag_z = 0;
% fault_status_flags_bad_mag_z = false;


%% rotate magnetometer earth field state into body frame

% R_to_body = Quat2Tbn(normQuat(states(1:4)));
mag_I = [magN;magE;magD];
R_to_body = quatToInverseRotMat(normQuat(states(1:4)));


mag_I_rot = R_to_body * mag_I;
% mag_I_rot =  mag_I;

% compute magnetometer innovations
mag_innov = mag_I_rot + mag_B - Measmag;

% Observation jacobian and Kalman gain vectors
% SparseVector24f<0,1,2,3,16,17,18,19,20,21> Hfusion;
% Vector24f Kfusion;
Hfusion = zeros(1,24);
Kfusion = zeros(24,1);

%% update the states and covariance using sequential fusion of the magnetometer components
for index = 1:3
	% Calculate Kalman gains and observation jacobians
	if (index == 1) 
		% Calculate X axis observation jacobians
		% Hfusion.at<0>() = 2*HKX0;
		% Hfusion.at<1>() = 2*HKX1;
		% Hfusion.at<2>() = 2*HKX2 - 2*HKX3 - 2*HKX4;
		% Hfusion.at<3>() = 2*HKX5;
		% Hfusion.at<16>() = HKX6;
		% Hfusion.at<17>() = 2*HKX7;
		% Hfusion.at<18>() = 2*HKX8 - 2*HKX9;
		% Hfusion.at<19>() = 1;
		Hfusion(1) = 2*HKX0;
		Hfusion(2) = 2*HKX1;
		Hfusion(3) = 2*HKX2 - 2*HKX3 - 2*HKX4;
		Hfusion(4) = 2*HKX5;
		Hfusion(17) = HKX6;
		Hfusion(18) = 2*HKX7;
		Hfusion(19) = 2*HKX8 - 2*HKX9;
		Hfusion(20) = 1;
		% Calculate X axis Kalman gains
		Kfusion(1) = HKX16*HKX24;
		Kfusion(2) = HKX22*HKX24;
		Kfusion(3) = HKX19*HKX24;
		Kfusion(4) = HKX21*HKX24;

		for row = 5:16
			Kfusion(row) = HKX24*(HKX10*P(row,18) - HKX11*P(row,19) + HKX12*P(2,row) + HKX13*P(1,row) - HKX14*P(3,row) + HKX15*P(4,row) + HKX6*P(row,17) + P(row,20));
        end

		for row = 23:24
			Kfusion(row) = HKX24*(HKX10*P(18,row) - HKX11*P(19,row) + HKX12*P(2,row) + HKX13*P(1,row) - HKX14*P(3,row) + HKX15*P(4,row) + HKX6*P(17,row) + P(20,row));
        end
    

		Kfusion(17) = HKX17*HKX24;
		Kfusion(18) = HKX20*HKX24;
		Kfusion(19) = HKX18*HKX24;
		Kfusion(20) = HKX23*HKX24;

		for row = 21:22
			Kfusion(row) = HKX24*(HKX10*P(18,row) - HKX11*P(19,row) + HKX12*P(2,row) + HKX13*P(1,row) - HKX14*P(3,row) + HKX15*P(4,row) + HKX6*P(17,row) + P(20,row));
        end

    elseif (index == 2) 

		% recalculate innovation variance becasue states and covariances have changed due to previous fusion
		HKY0 = magD*q1 + magE*q0 - magN*q3;
		HKY1 = magD*q0 - magE*q1 + magN*q2;
		HKY2 = magD*q3 + magE*q2 + magN*q1;
		HKY3 = magD*q2;
		HKY4 = magE*q3;
		HKY5 = magN*q0;
		HKY6 = q1*q2;
		HKY7 = q0*q3;
		HKY8 = power(q0, 2) - power(q1, 2) + power(q2, 2) - power(q3, 2);
		HKY9 = q0*q1 + q2*q3;
		HKY10 = 2*HKY9;
		HKY11 = -2*HKY6 + 2*HKY7;
		HKY12 = 2*HKY2;
		HKY13 = 2*HKY0;
		HKY14 = 2*HKY1;
		HKY15 = -2*HKY3 + 2*HKY4 + 2*HKY5;
	  % HKY16 = HKY10*P(0,18) - HKY11*P(0,16) + HKY12*P(0,2) + HKY13*P(0,0) + HKY14*P(0,1) - HKY15*P(0,3) + HKY8*P(0,17) + P(0,20);
		HKY16 = HKY10*P(1,19) - HKY11*P(1,17) + HKY12*P(1,3) + HKY13*P(1,1) + HKY14*P(1,2) - HKY15*P(1,4) + HKY8*P(1,18) + P(1,21);
	  % HKY17 = HKY10*P(17,18) - HKY11*P(16,17) + HKY12*P(2,17) + HKY13*P(0,17) + HKY14*P(1,17) - HKY15*P(3,17) + HKY8*P(17,17) + P(17,20);
        HKY17 = HKY10*P(18,19) - HKY11*P(17,18) + HKY12*P(3,18) + HKY13*P(1,18) + HKY14*P(2,18) - HKY15*P(4,18) + HKY8*P(18,18) + P(18,21);
	  % HKY18 = HKY10*P(16,18) - HKY11*P(16,16) + HKY12*P(2,16) + HKY13*P(0,16) + HKY14*P(1,16) - HKY15*P(3,16) + HKY8*P(16,17) + P(16,20);
		HKY18 = HKY10*P(17,19) - HKY11*P(17,17) + HKY12*P(3,17) + HKY13*P(4,17) + HKY14*P(2,17) - HKY15*P(4,17) + HKY8*P(17,18) + P(17,21);
	  % HKY19 = HKY10*P(3,18) - HKY11*P(3,16) + HKY12*P(2,3) + HKY13*P(0,3) + HKY14*P(1,3) - HKY15*P(3,3) + HKY8*P(3,17) + P(3,20);
		HKY19 = HKY10*P(4,19) - HKY11*P(4,17) + HKY12*P(3,4) + HKY13*P(1,4) + HKY14*P(2,4) - HKY15*P(4,4) + HKY8*P(4,18) + P(4,21);
      % HKY20 = HKY10*P(18,18) - HKY11*P(16,18) + HKY12*P(2,18) + HKY13*P(0,18) + HKY14*P(1,18) - HKY15*P(3,18) + HKY8*P(17,18) + P(18,20);
		HKY20 = HKY10*P(19,19) - HKY11*P(17,19) + HKY12*P(3,19) + HKY13*P(1,19) + HKY14*P(2,19) - HKY15*P(4,19) + HKY8*P(18,19) + P(19,21);
      % HKY21 = HKY10*P(1,18) - HKY11*P(1,16) + HKY12*P(1,2) + HKY13*P(0,1) + HKY14*P(1,1) - HKY15*P(1,3) + HKY8*P(1,17) + P(1,20);
		HKY21 = HKY10*P(2,19) - HKY11*P(2,17) + HKY12*P(2,3) + HKY13*P(1,2) + HKY14*P(2,2) - HKY15*P(2,4) + HKY8*P(2,18) + P(2,21);
      % HKY22 = HKY10*P(2,18) - HKY11*P(2,16) + HKY12*P(2,2) + HKY13*P(0,2) + HKY14*P(1,2) - HKY15*P(2,3) + HKY8*P(2,17) + P(2,20);
		HKY22 = HKY10*P(3,19) - HKY11*P(3,17) + HKY12*P(3,3) + HKY13*P(1,3) + HKY14*P(2,3) - HKY15*P(3,4) + HKY8*P(3,18) + P(3,21);
      % HKY23 = HKY10*P(18,20) - HKY11*P(16,20) + HKY12*P(2,20) + HKY13*P(0,20) + HKY14*P(1,20) - HKY15*P(3,20) + HKY8*P(17,20) + P(20,20);
		HKY23 = HKY10*P(19,21) - HKY11*P(17,21) + HKY12*P(3,21) + HKY13*P(1,21) + HKY14*P(2,21) - HKY15*P(4,21) + HKY8*P(18,21) + P(21,21);
		mag_innov_var(2) = (HKY10*HKY20 - HKY11*HKY18 + HKY12*HKY22 + HKY13*HKY16 + HKY14*HKY21 - HKY15*HKY19 + HKY17*HKY8 + HKY23 + R_MAG);

        if (mag_innov_var(2) < R_MAG) 
	        % the innovation variance contribution from the state covariances is negative which means the covariance matrix is badly conditioned
	        fault_status_flags_bad_mag_y = 1;
        
	        % we need to re-initialise covariances and abort this fusion step
	        % resetMagRelatedCovariances();
            P = resetMagRelatedCovariances(P,states);
            return;
        end       
		HKY24 = 1.0/mag_innov_var(2);

		%% Calculate Y axis observation jacobians
		Hfusion = zeros(1,24);
		Hfusion(1) = 2*HKY0;
		Hfusion(2) = 2*HKY1;
		Hfusion(3) = 2*HKY2;
		Hfusion(4) = 2*HKY3 - 2*HKY4 - 2*HKY5;
		Hfusion(17) = 2*HKY6 - 2*HKY7;
		Hfusion(18) = HKY8;
		Hfusion(19) = 2*HKY9;
		Hfusion(21) = 1;

		%Calculate Y axis Kalman gains
		Kfusion(1) = HKY16*HKY24;
		Kfusion(2) = HKY21*HKY24;
		Kfusion(3) = HKY22*HKY24;
		Kfusion(4) = HKY19*HKY24;

		for row = 5:16
			Kfusion(row) = HKY24*(HKY10*P(row,19) - HKY11*P(row,17) + HKY12*P(3,row) + HKY13*P(1,row) + HKY14*P(2,row) - HKY15*P(4,row) + HKY8*P(row,18) + P(row,21));
        end

		for row = 23:24
			Kfusion(row) = HKY24*(HKY10*P(19,row) - HKY11*P(17,row) + HKY12*P(3,row) + HKY13*P(1,row) + HKY14*P(2,row) - HKY15*P(4,row) + HKY8*P(18,row) + P(21,row));
        end
	

		Kfusion(17) = HKY18*HKY24;
		Kfusion(18) = HKY17*HKY24;
		Kfusion(19) = HKY20*HKY24;
		Kfusion(20) = HKY24*(HKY10*P(19,20) - HKY11*P(17,20) + HKY12*P(3,20) + HKY13*P(1,20) + HKY14*P(2,20) - HKY15*P(4,20) + HKY8*P(18,20) + P(20,21));
		Kfusion(21) = HKY23*HKY24;
		Kfusion(22) = HKY24*(HKY10*P(19,22) - HKY11*P(17,22) + HKY12*P(3,22) + HKY13*P(1,22) + HKY14*P(2,22) - HKY15*P(4,22) + HKY8*P(18,22) + P(21,22));

    elseif (index == 3) 
		
        % recalculate innovation variance becasue states and covariances have changed due to previous fusion
		HKZ0 = magD*q0 - magE*q1 + magN*q2;
		HKZ1 = magN*q3;
		HKZ2 = magD*q1;
		HKZ3 = magE*q0;
		HKZ4 = -magD*q2 + magE*q3 + magN*q0;
		HKZ5 = magD*q3 + magE*q2 + magN*q1;
		HKZ6 = q0*q2 + q1*q3;
		HKZ7 = q2*q3;
		HKZ8 = q0*q1;
		HKZ9 = power(q0, 2) - power(q1, 2) - power(q2, 2) + power(q3, 2);
		HKZ10 = 2*HKZ6;
		HKZ11 = -2*HKZ7 + 2*HKZ8;
		HKZ12 = 2*HKZ5;
		HKZ13 = 2*HKZ0;
		HKZ14 = -2*HKZ1 + 2*HKZ2 + 2*HKZ3;
		HKZ15 = 2*HKZ4;
	  % HKZ16 = HKZ10*P(0,16) - HKZ11*P(0,17) + HKZ12*P(0,3) + HKZ13*P(0,0) - HKZ14*P(0,1) + HKZ15*P(0,2) + HKZ9*P(0,18) + P(0,21);
		HKZ16 = HKZ10*P(1,17) - HKZ11*P(1,18) + HKZ12*P(1,4) + HKZ13*P(1,1) - HKZ14*P(1,2) + HKZ15*P(1,3) + HKZ9*P(1,19) + P(1,22);
      % HKZ17 = HKZ10*P(16,18) - HKZ11*P(17,18) + HKZ12*P(3,18) + HKZ13*P(0,18) - HKZ14*P(1,18) + HKZ15*P(2,18) + HKZ9*P(18,18) + P(18,21);
        HKZ17 = HKZ10*P(17,19) - HKZ11*P(18,19) + HKZ12*P(4,19) + HKZ13*P(1,19) - HKZ14*P(2,19) + HKZ15*P(3,19) + HKZ9*P(19,19) + P(19,22);
      % HKZ18 = HKZ10*P(16,17) - HKZ11*P(17,17) + HKZ12*P(3,17) + HKZ13*P(0,17) - HKZ14*P(1,17) + HKZ15*P(2,17) + HKZ9*P(17,18) + P(17,21);
		HKZ18 = HKZ10*P(17,18) - HKZ11*P(18,18) + HKZ12*P(4,18) + HKZ13*P(1,18) - HKZ14*P(2,18) + HKZ15*P(3,18) + HKZ9*P(18,19) + P(18,22);
      % HKZ19 = HKZ10*P(1,16) - HKZ11*P(1,17) + HKZ12*P(1,3) + HKZ13*P(0,1) - HKZ14*P(1,1) + HKZ15*P(1,2) + HKZ9*P(1,18) + P(1,21);
		HKZ19 = HKZ10*P(2,17) - HKZ11*P(2,18) + HKZ12*P(2,4) + HKZ13*P(1,2) - HKZ14*P(2,2) + HKZ15*P(2,3) + HKZ9*P(2,19) + P(2,22);
      % HKZ20 = HKZ10*P(16,16) - HKZ11*P(16,17) + HKZ12*P(3,16) + HKZ13*P(0,16) - HKZ14*P(1,16) + HKZ15*P(2,16) + HKZ9*P(16,18) + P(16,21);
		HKZ20 = HKZ10*P(17,17) - HKZ11*P(17,18) + HKZ12*P(4,17) + HKZ13*P(4,17) - HKZ14*P(2,17) + HKZ15*P(3,17) + HKZ9*P(17,19) + P(17,22);
      % HKZ21 = HKZ10*P(3,16) - HKZ11*P(3,17) + HKZ12*P(3,3) + HKZ13*P(0,3) - HKZ14*P(1,3) + HKZ15*P(2,3) + HKZ9*P(3,18) + P(3,21);
		HKZ21 = HKZ10*P(4,17) - HKZ11*P(4,18) + HKZ12*P(4,4) + HKZ13*P(1,4) - HKZ14*P(2,4) + HKZ15*P(3,4) + HKZ9*P(4,19) + P(4,22);
      % HKZ22 = HKZ10*P(2,16) - HKZ11*P(2,17) + HKZ12*P(2,3) + HKZ13*P(0,2) - HKZ14*P(1,2) + HKZ15*P(2,2) + HKZ9*P(2,18) + P(2,21);
		HKZ22 = HKZ10*P(3,17) - HKZ11*P(3,18) + HKZ12*P(3,4) + HKZ13*P(1,3) - HKZ14*P(2,4) + HKZ15*P(3,3) + HKZ9*P(3,19) + P(3,22);
      % HKZ23 = HKZ10*P(16,21) - HKZ11*P(17,21) + HKZ12*P(3,21) + HKZ13*P(0,21) - HKZ14*P(1,21) + HKZ15*P(2,21) + HKZ9*P(18,21) + P(21,21);
		HKZ23 = HKZ10*P(17,22) - HKZ11*P(18,22) + HKZ12*P(4,22) + HKZ13*P(1,22) - HKZ14*P(2,22) + HKZ15*P(3,22) + HKZ9*P(19,22) + P(22,22);

        if (mag_innov_var(3) < R_MAG) 
	        % the innovation variance contribution from the state covariances is negative which means the covariance matrix is badly conditioned
	        fault_status_flags_bad_mag_z = 1;
        
	        % we need to re-initialise covariances and abort this fusion step
	        % resetMagRelatedCovariances();
            P = resetMagRelatedCovariances(P,states);
            return;
        end

		mag_innov_var(3) = (HKZ10*HKZ20 - HKZ11*HKZ18 + HKZ12*HKZ21 + HKZ13*HKZ16 - HKZ14*HKZ19 + HKZ15*HKZ22 + HKZ17*HKZ9 + HKZ23 + R_MAG);

		HKZ24 = 1.0/mag_innov_var(3);

		% calculate Z axis observation jacobians
		Hfusion = zeros(1,24);
		Hfusion(1) = 2*HKZ0;
		Hfusion(2) = 2*HKZ1 - 2*HKZ2 - 2*HKZ3;
		Hfusion(3) = 2*HKZ4;
		Hfusion(4) = 2*HKZ5;
		Hfusion(17) = 2*HKZ6;
		Hfusion(18) = 2*HKZ7 - 2*HKZ8;
		Hfusion(19) = HKZ9;
		Hfusion(22) = 1;

		% Calculate Z axis Kalman gains
		Kfusion(1) = HKZ16*HKZ24;
		Kfusion(2) = HKZ19*HKZ24;
		Kfusion(3) = HKZ22*HKZ24;
		Kfusion(4) = HKZ21*HKZ24;

		for row = 5:16 
            % Kfusion(row) = HKZ24*(HKZ10*P(row,16) - HKZ11*P(row,17) + HKZ12*P(3,row) + HKZ13*P(0,row) - HKZ14*P(1,row) + HKZ15*P(2,row) + HKZ9*P(row,18) + P(row,21));
            Kfusion(row) = HKZ24*(HKZ10*P(row,17) - HKZ11*P(row,18) + HKZ12*P(4,row) + HKZ13*P(1,row) - HKZ14*P(2,row) + HKZ15*P(3,row) + HKZ9*P(row,19) + P(row,22));
        end

		for row = 23:24
		  % Kfusion(row) = HKZ24*(HKZ10*P(16,row) - HKZ11*P(17,row) + HKZ12*P(3,row) + HKZ13*P(0,row) - HKZ14*P(1,row) + HKZ15*P(2,row) + HKZ9*P(18,row) + P(21,row));
            Kfusion(row) = HKZ24*(HKZ10*P(17,row) - HKZ11*P(18,row) + HKZ12*P(4,row) + HKZ13*P(1,row) - HKZ14*P(2,row) + HKZ15*P(3,row) + HKZ9*P(19,row) + P(22,row));
        end


		Kfusion(17) = HKZ20*HKZ24;
		Kfusion(18) = HKZ18*HKZ24;
		Kfusion(19) = HKZ17*HKZ24;

		for row = 20:21
		  % Kfusion(row) = HKZ24*(HKZ10*P(16,row) - HKZ11*P(17,row) + HKZ12*P(3,row) + HKZ13*P(0,row) - HKZ14*P(1,row) + HKZ15*P(2,row) + HKZ9*P(18,row) + P(row,21));
			Kfusion(row) = HKZ24*(HKZ10*P(17,row) - HKZ11*P(18,row) + HKZ12*P(4,row) + HKZ13*P(1,row) - HKZ14*P(2,row) + HKZ15*P(3,row) + HKZ9*P(19,row) + P(row,22));
            
        end

		Kfusion(22) = HKZ23*HKZ24;
    end

%% is_fused = measurementUpdate(Kfusion, Hfusion, mag_innov(index));
    
    KHP = computeKHP(P,Kfusion, Hfusion);
	for i = 1:24
		if (P(i, i) < KHP(i, i)) 
			% P.uncorrelateCovarianceSetVariance<1>(i, 0.0f);
			healthy = 0;
            P = single(zeros(24,24));
            return;
        end
	end
    P= P- KHP;
    % fixCovarianceErrors(true);
    P = fixCovarianceErrors(P,1);
    states = states - Kfusion*mag_innov(index);
    fault_status_flags_bad_mag = [fault_status_flags_bad_mag_x,fault_status_flags_bad_mag_y,fault_status_flags_bad_mag_z];
    % limitDeclination();
end


end
